simulink model "ElectricalCoupling_testing"  (R2024b)
settings: Solver=FixedStepAuto  StartTime=0.0  StopTime=20  RelTol=1e-3
undefined symbols (not defined in the file): ac4b, c4e6, DiscIntNeverNeededParam
libraries: fl_lib x22, nesl_utility x21, ee_lib x5, simulink x3
(part 1 of 2)
settings Model: Creator=rodri  LastModifiedBy=rodri
settings SolverCC: ConcurrentTasks=on  PositivePriorityOrder=on
settings OptimizationCC: BlockReduction=off  OptimizeBlockIOStorage=off
settings DebuggingCC: TasksWithSamePriorityMsg=none
settings HardwareCC: ProdBitPerLong=64  ProdLongLongMode=on  ProdHWDeviceType=Intel->x86-64 (Linux 64)
settings RTWCC: Description=Simulink Real-Time  SystemTargetFile=slrealtime.tlc  TemplateMakefile=slrealtime_default_tmf  Toolchain=Simulink Real-Time Toolchain  BuildConfiguration=Faster Runs  CodeExecutionProfiling=on  TargetLang=C++  GPUComputeCapability=3.5
settings SimulinkRealTimeTargetCC: InstructionSetFMA=off  LogToMDFFile=off

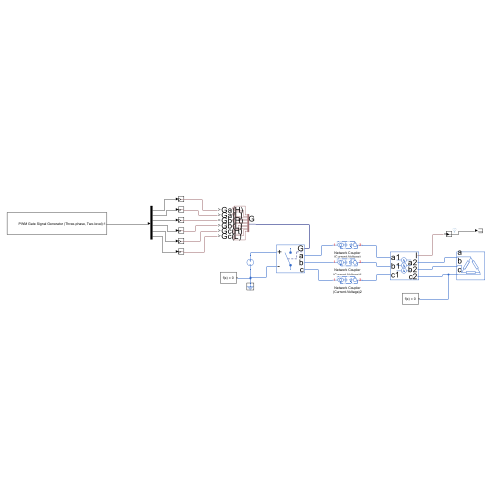
[thumbnail: Simulink's stored preview of the top-level diagram]
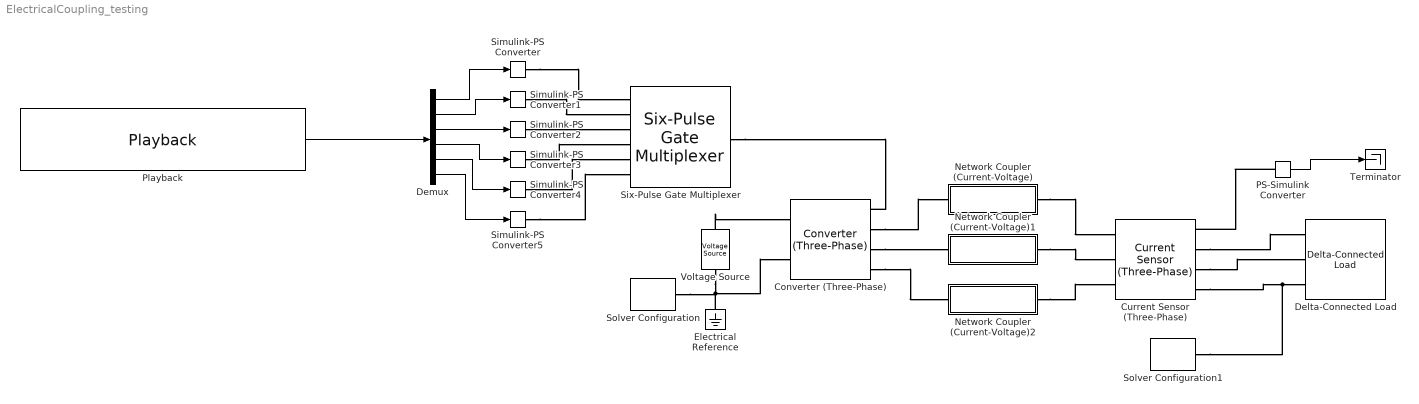
== system ElectricalCoupling_testing ==
  Converter (Three-Phase) : ee_lib/Semiconductors & Converters/Converters/Converter (Three-Phase)  port_option=ee.enum.threePhasePort.expanded  fidelity_option=ee.enum.converters.fidelity.detailed  device_type=ee.enum.converters.switchingdevice.ideal  showThermalPort=false  K=0  Vth=0.5 V  Vgt=1 V  Vgt_off=-1 V  Ih=1 A  Vf=0.8 V  Ron=0.001 Ohm  Rds=0.001 Ohm  Goff=1e-6 1/Ohm  Eon_scalar=22.86e-3 J  Eoff_scalar=17.14e-3 J  Eoff_natural_commutation=10e-3 J  Voff=300 V  Iout_scalar=600 A  onCurrentMeasDelay=0 s  useCurrentFromPreviousCycle=false  useVoltageFromPreviousCycle=false  diode_param=ee.enum.converters.protectiondiode.none  diode_Vf=0.8 V  diode_Ron=0.001 Ohm  diode_Goff=1e-5 1/Ohm  diode_C=50 nF  diode_iRM=-235 A  diode_iF=300 A  diode_idot=-50 A/us  diode_trr_param=ee.enum.converters.diodetrr.trr_factor  diode_trr_factor=3  diode_trr=15 us  diode_Qrr=1500 s*uA  diode_rec_loss_model=ee.enum.diode.reverseRecoveryModel.fixed  diode_ErecVal=0 J  diode_scaleWithIandV=false  diode_ErecMat=zeros(2, 3) J  diode_TjrecVec=[298.15, 398.15] K  diode_IfrecVec=[.1, 1, 10] A  diode_IrecVal=10 A  diode_VrecVal=10 V  diode_tFilter=1 / 1000 / 100 s  thermal_network_parameterization=ee.enum.thermalNetworkTopology.external  Rth=[.08, .5] K/W  Rth_Cauer=[.08, .1, .5] K/W  Rth_Foster=[.08, .14, .22, .16] K/W  thermal_mass_parameterization=ee.enum.thermalNetwork.timeconstant  thermal_mass=[.01, .5] J/K  thermal_mass_Cauer=[.01, .1, .5] J/K  thermal_mass_Foster=[.001, .005, .05, .5] J/K  thermal_time_constant=[.001, .2] s  thermal_time_constant_Cauer=[.001, .1, .2] s  thermal_time_constant_Foster=[7e-05, .0007, .01, .08] s  thermal_mass_initial_temperatures=[25, 25] degC  thermal_mass_initial_temperatures_Cauer=[25, 25, 25] degC  junction_thermal_mass=0.01 J/K  Tvec_initial_Foster=[25, 25, 25, 25] degC  snubber_type=ee.enum.converters.snubber.exclude  Cs=1e-7 F  Rs=0.1 Ohm  Vce_loss=[0, 150, 300] V
      settings: InternalSimscapePortConfiguration="{\"Bottom\":[],\"Left\":[{\"id\":\"G\",\"label\":\"G\",\"type\":\"foundation.electrical.twelve_phase\"},{\"id\":\"a\",\"label\":\"a\",\"type\":\"foundation.electrical.electrical\"},{\"id\":\"b\",\"label\":\"b\",\"type\":\"foundation.electrical.electrical\"},{\"id\":\"c\",\"label\":\"c\",\"type\":\"foundation.electrical.electrical\"}],\"Right\":[{\"id\":\"p\",\"label\":\"+\",\"type\":\"foundation.electrical.electrical\"},{\"id\":\"n\",\"label\":\"-\",\"type\":\"foundation.electrical.electrical\"}],\"Top\":[]}"
  Current Sensor (Three-Phase) : ee_lib/Sensors & Transducers/Current Sensor (Three-Phase)
      settings: InternalSimscapePortConfiguration="{\"Bottom\":[],\"Left\":[{\"id\":\"a1\",\"label\":\"a1\",\"type\":\"foundation.electrical.electrical\"},{\"id\":\"b1\",\"label\":\"b1\",\"type\":\"foundation.electrical.electrical\"},{\"id\":\"c1\",\"label\":\"c1\",\"type\":\"foundation.electrical.electrical\"}],\"Right\":[{\"id\":\"I_output\",\"label\":\"I\",\"type\":\"output\"},{\"id\":\"a2\",\"label\":\"a2\",\"type\":\"foundation.electrical.electrical\"},{\"id\":\"b2\",\"label\":\"b2\",\"type\":\"foundation.electrical.electrical\"},{\"id\":\"c2\",\"label\":\"c2\",\"type\":\"foundation.electrical.electrical\"}],\"Top\":[]}"
  Delta-Connected Load : ee_lib/Passive/RLC Assemblies/Delta-Connected Load  port_option=ee.enum.threePhasePort.expanded  parameterization=ee.enum.rlc.parameterization.ratedpower  component_structure=ee.enum.rlc.structure.R  component_structure_PQ=ee.enum.rlc.structure.SeriesRL  R=1 Ohm  L=1e-3 H  C=1e-6 F  VRated=380 V  FRated=60 Hz  P=10e3 W  Qpos=1e3 A*V  Qneg=-1e2 A*V  R_parasitic=0 Ohm  G_parasitic=0 1/Ohm  R_parasitic_PQ=0 Ohm  G_parasitic_PQ=0 1/Ohm  Vmag0=0 V  Vang0=0 deg  Freq0=60 Hz  IL_specify=off  IL_priority=High  IL=[0, 0, 0] A  IL_nominal_specify=off  IL_nominal_value=1  IL_nominal_unit=A  VC_specify=off  VC_priority=High  VC=[0, 0, 0] V  VC_nominal_specify=off  VC_nominal_value=1  VC_nominal_unit=V
      settings: InternalSimscapePortConfiguration="{\"Bottom\":[],\"Left\":[{\"id\":\"a\",\"label\":\"a\",\"type\":\"foundation.electrical.electrical\"},{\"id\":\"b\",\"label\":\"b\",\"type\":\"foundation.electrical.electrical\"},{\"id\":\"c\",\"label\":\"c\",\"type\":\"foundation.electrical.electrical\"}],\"Right\":[],\"Top\":[]}"
  Demux : Demux  Outputs=6
  Electrical Reference : fl_lib/Electrical/Electrical Elements/Electrical Reference
  Network Coupler (Current-Voltage) : Subsystem  mask(Network Coupler (Current-Voltage)){}
      mask init:
      | % Icon
      | key = 'Simscape.NetworkCouplers.ElectricalCurrentVoltage';
      | foundation.internal.couplers.updateIcon(gcb,'currentVoltageSource.svg',key)
      settings: OpenFcn=open_system(gcbh,'force')
      mask Help: web([docroot '/simscape/ref/networkcouplercurrentvoltage.html'])
      mask Display:
      | color('red');
      | port_label('LConn', 1,'1')
      | port_label('RConn', 1,'2')
  Network Coupler (Current-Voltage)1 : Subsystem  mask(Network Coupler (Current-Voltage)){}
      mask init:
      | % Icon
      | key = 'Simscape.NetworkCouplers.ElectricalCurrentVoltage';
      | foundation.internal.couplers.updateIcon(gcb,'currentVoltageSource.svg',key)
      settings: OpenFcn=open_system(gcbh,'force')
      mask Help: web([docroot '/simscape/ref/networkcouplercurrentvoltage.html'])
      mask Display:
      | color('red');
      | port_label('LConn', 1,'1')
      | port_label('RConn', 1,'2')
  Network Coupler (Current-Voltage)2 : Subsystem  mask(Network Coupler (Current-Voltage)){}
      mask init:
      | % Icon
      | key = 'Simscape.NetworkCouplers.ElectricalCurrentVoltage';
      | foundation.internal.couplers.updateIcon(gcb,'currentVoltageSource.svg',key)
      settings: OpenFcn=open_system(gcbh,'force')
      mask Help: web([docroot '/simscape/ref/networkcouplercurrentvoltage.html'])
      mask Display:
      | color('red');
      | port_label('LConn', 1,'1')
      | port_label('RConn', 1,'2')
  PS-Simulink Converter : nesl_utility/PS-Simulink Converter  PhysicalDomain=network_engine_domain  SubClassName=ps_output  LeftPortType=input  RightPortType=output  PseudoPeriodic=off  Frequencies=[]  VectorFormat=inherit  Unit=inherit  AffineConversion=off
  Playback : Playback  NumPorts=1  PartName=31bf6123-c4e6-46bc-ac4b-6301b38411a2
  Simulink-PS Converter{,1..5} (6 alike) : nesl_utility/Simulink-PS Converter  PhysicalDomain=network_engine_domain  SubClassName=ps_input  LeftPortType=input  RightPortType=output  PseudoPeriodic=off  Frequencies=[]  NoiseDistribution=none  NoiseParameters=[]  Unit=1  AffineConversion=off  FilteringAndDerivatives=provide  SimscapeFilterOrder=1  InputFilterTimeConstant=0.001  UdotUserProvided=0
  Six-Pulse Gate Multiplexer : ee_lib/Semiconductors & Converters/Converters/Six-Pulse Gate Multiplexer  port_option=ee.enum.controlport.ps
  Solver Configuration : nesl_utility/Solver Configuration  PhysicalDomain=network_engine_domain  SubClassName=solver  LeftPortType=input  RightPortType=generic  Tones=[]  Harmonics=[]  SimulateNoise=off  Profile=off  UseLocalSampling=off  EnableSwitchedLinearOptims=on  FrequencyDomain=off  UseCCode=off  RelTol=0.001  AbsTol=0.001  MinStep=1e-09  ToWorkspace=off  RevertToSquareIcSolve=off  NumHomotopyIterations=100  PhasorMode=off  PhasorModeNumHarmonics=1  ConsistencySolver=NEWTON_XTOL_AFTER_FTOL  IndexReductionMethod=DerivativeReplacement  DoDC=off  ResidualTolerance=1e-09  ConsistencyTolSource=GLOBAL  ConsistencyAbsTol=0.001  ConsistencyRelTol=0.001  ConsistencyTolFactor=0.001  UseLocalSolver=off  LocalSolverChoice=NE_BACKWARD_EULER_ADVANCER  ResolveIndetEquations=on  FunctionEvalNumThread=1  LocalSolverSampleTime=0.001  DoFixedCost=off  MaxNonlinIter=3  MaxModeIter=2  ComputeImpulses=off  ImpulseIterations=2  LinearAlgebra=auto  LinearAlgebraNumThread=0  EquationFormulation=NE_TIME_EF  DelaysMemoryBudget=1024  AutomaticFiltering=on  FilteringTimeConstant=0.001  PartitionStorageMethod=AS_NEEDED  PartitionMemoryBudget=1024  PartitionMethod=ROBUST  MultibodyUseLocalSolver=off  MultibodyLocalSolverChoice=ODE1  MultibodyLocalSolverSampleTime=0.001
  Solver Configuration1 : nesl_utility/Solver Configuration  PhysicalDomain=network_engine_domain  SubClassName=solver  LeftPortType=input  RightPortType=generic  Tones=[]  Harmonics=[]  SimulateNoise=off  Profile=off  UseLocalSampling=off  EnableSwitchedLinearOptims=on  FrequencyDomain=off  UseCCode=off  RelTol=0.001  AbsTol=0.001  MinStep=1e-09  ToWorkspace=off  RevertToSquareIcSolve=off  NumHomotopyIterations=100  PhasorMode=off  PhasorModeNumHarmonics=1  ConsistencySolver=NEWTON_XTOL_AFTER_FTOL  IndexReductionMethod=DerivativeReplacement  DoDC=off  ResidualTolerance=1e-09  ConsistencyTolSource=GLOBAL  ConsistencyAbsTol=0.001  ConsistencyRelTol=0.001  ConsistencyTolFactor=0.001  UseLocalSolver=off  LocalSolverChoice=NE_BACKWARD_EULER_ADVANCER  ResolveIndetEquations=on  FunctionEvalNumThread=1  LocalSolverSampleTime=0.001  DoFixedCost=off  MaxNonlinIter=3  MaxModeIter=2  ComputeImpulses=off  ImpulseIterations=2  LinearAlgebra=auto  LinearAlgebraNumThread=0  EquationFormulation=NE_TIME_EF  DelaysMemoryBudget=1024  AutomaticFiltering=on  FilteringTimeConstant=0.001  PartitionStorageMethod=AS_NEEDED  PartitionMemoryBudget=1024  PartitionMethod=ROBUST  MultibodyUseLocalSolver=off  MultibodyLocalSolverChoice=ODE1  MultibodyLocalSolverSampleTime=0.001
  Terminator : Terminator
  Voltage Source : ee_lib/Sources/Voltage Source  dc_voltage=380 V  ac_voltage=0 V  ac_shift=0 rad  ac_frequency=60 Hz  noise_mode=ee.enum.sources.noise.Disabled  PSD=0 V^2/Hz  sample_time=1e-3 s  repeatability=ee.enum.sources.repeatability.NotRepeatable  user_seed=0  auto_seed=3499211588  i_specify=off  i_priority=None  i=0 A  i_nominal_specify=off  i_nominal_value=1  i_nominal_unit=A  v_specify=off  v_priority=None  v=0 V  v_nominal_specify=off  v_nominal_value=1  v_nominal_unit=V
  wires:
  Demux/1 -> Simulink-PS Converter/1
  Demux/2 -> Simulink-PS Converter1/1
  Demux/3 -> Simulink-PS Converter2/1
  Demux/4 -> Simulink-PS Converter3/1
  Demux/5 -> Simulink-PS Converter4/1
  Demux/6 -> Simulink-PS Converter5/1
  Playback/1 -> Demux/1
  PS-Simulink Converter/1 -> Terminator/1
  connections:
  Simulink-PS Converter2/RConn1 -- Six-Pulse Gate Multiplexer/LConn3
  Simulink-PS Converter1/RConn1 -- Six-Pulse Gate Multiplexer/LConn2
  Simulink-PS Converter3/RConn1 -- Six-Pulse Gate Multiplexer/LConn4
  Simulink-PS Converter/RConn1 -- Six-Pulse Gate Multiplexer/LConn1
  Simulink-PS Converter4/RConn1 -- Six-Pulse Gate Multiplexer/LConn5
  Simulink-PS Converter5/RConn1 -- Six-Pulse Gate Multiplexer/LConn6
  Six-Pulse Gate Multiplexer/RConn1 -- Converter (Three-Phase)/LConn1
  Voltage Source/LConn1 -- Converter (Three-Phase)/RConn1
  Voltage Source/RConn1 -- Solver Configuration/RConn1 -- Electrical Reference/LConn1 -- Converter (Three-Phase)/RConn2
  Current Sensor (Three-Phase)/RConn2 -- Delta-Connected Load/LConn1
  PS-Simulink Converter/LConn1 -- Current Sensor (Three-Phase)/RConn1
  Converter (Three-Phase)/LConn2 -- Network Coupler (Current-Voltage)/LConn1
  Network Coupler (Current-Voltage)/RConn1 -- Current Sensor (Three-Phase)/LConn1
  Network Coupler (Current-Voltage)1/RConn1 -- Current Sensor (Three-Phase)/LConn2
  Converter (Three-Phase)/LConn3 -- Network Coupler (Current-Voltage)1/LConn1
  Converter (Three-Phase)/LConn4 -- Network Coupler (Current-Voltage)2/LConn1
  Network Coupler (Current-Voltage)2/RConn1 -- Current Sensor (Three-Phase)/LConn3
  Current Sensor (Three-Phase)/RConn4 -- Solver Configuration1/RConn1 -- Delta-Connected Load/LConn3
  Current Sensor (Three-Phase)/RConn3 -- Delta-Connected Load/LConn2

== system ElectricalCoupling_testing/Network Coupler (Current-Voltage) ==
  note: Connect Port 1 to the network
      | with the smaller sample time, or
      | the network running variable step.
  note: Uncomment rate transition
      | blocks if one or both networks
      | are running fixed step.
  Port 1 Interface : Subsystem  mask(Network Coupler (Current-Voltage) Port 1 Interface){samplingType=Variable step at ports 1 and 2, ts=1e-3, h1=0.0002, h2=0.001, predictionDiscreteToContinuous=off, smoothingContinuousToDiscrete=off, predictionSlowToFast=off, smoothingFastToSlow=off, nSmooth=1, tsSmoothing=0.01, tsMax=0.005, tau=0.001, i0=0, v0=0}
      mask prompts: samplingType "physmod:simscape:couplers:SimscapeNetworkCouplersLib:SamplingType_MP"; ts "physmod:simscape:couplers:SimscapeNetworkCouplersLib:SeparatorTimeConstants_MP"; h1 "physmod:simscape:couplers:SimscapeNetworkCouplersLib:Port1NetworkDiscreteSampleTimes_MP"; h2 "physmod:simscape:couplers:SimscapeNetworkCouplersLib:Port2NetworkDiscreteSampleTimes_MP"; predictionDiscreteToContinuous "physmod:simscape:couplers:SimscapeNetworkCouplersLib:UsePredictionWhenConnectingFixedStepToVariableStep_MP"; smoothingContinuousToDiscrete "physmod:simscape:couplers:SimscapeNetworkCouplersLib:UseSmoothingWhenConnectingVariableStepToFixedStep_MP"; predictionSlowToFast "physmod:simscape:couplers:SimscapeNetworkCouplersLib:UsePredictionWhenConnectingSlowToFastSampleTimes_MP"; smoothingFastToSlow "physmod:simscape:couplers:SimscapeNetworkCouplersLib:UseSmoothingWhenConnectingFastToSlowSampleTimes_MP"; nSmooth "physmod:simscape:couplers:SimscapeNetworkCouplersLib:NumberOfSamplesOverWhichToSmooth_MP"; tsSmoothing "physmod:simscape:couplers:SimscapeNetworkCouplersLib:SmoothingTimeConstants_MP"; tsMax "physmod:simscape:couplers:SimscapeNetworkCouplersLib:CalculatedFastestTrackableTimeConstants_MP"; tau "physmod:simscape:couplers:SimscapeNetworkCouplersLib:CalculatedFilterTimeConstants_MP"; i0 "physmod:simscape:couplers:SimscapeNetworkCouplersLib:InitialCurrentA_MP"; v0 "physmod:simscape:couplers:SimscapeNetworkCouplersLib:InitialVoltageV_MP"
      mask help: physmod:simscape:couplers:SimscapeNetworkCouplersLib:NetworkCouplerCurrentVoltagePort1Interface_MD
      mask init:
      | % Fixed step sample time value check
      | foundation.internal.couplers.checkSampleTimes(gcb,h1,h2);
      | 
      | % Derived parameters
      | [tau,tsMax] = foundation.internal.couplers.electrical.derivedParamsSources(gcb,ts,h1,h2);
      settings: PortSchema="{\"entries\":[{\"content\":{\"sides\":[{\"content\":{\"connectorIds\":[\"LConn1\"]},\"type\":\"ConnectorPlacement.EquallySpacedRectSide\",\"uuid\":\"a6d4a9fd-b5aa-40dc-ab7e-2b646b9b57bc\"},{\"content\":{\"connectorIds\":[\"Out1\",\"In1\"],\"side\":\"RIGHT\"},\"type\":\"ConnectorPlacement.EquallySpacedRectSide\",\"uuid\":\"31bb6273-5b9b-48d0-a1a2-6fbacb979b97\"},{\"content\":{\"connectorIds\":[],\"side\":\"TOP\"},\"type\":\"ConnectorPlacement.EquallySpacedRectSide\",\"uuid\":\"0f7afab2-4481-486c-9ad0-2b42c5b091a4\"}]},\"type\":\"ConnectorPlacement.EquallySpacedConnector\",\"uuid\":\"a98e47aa-cbfd-441a-b14c-c9ea515c056e\"}],\"packageUris\":[\"http://schema.mathworks.com/mf0/Connector/R2020b\"],\"version\":\"1.0\"}"
      mask Help: web([docroot '/simscape/ref/networkcouplercurrentvoltage.html'])
      mask TypeOptions samplingType: physmod:simscape:couplers:SimscapeNetworkCouplersLib:VariableStepAtPorts1And2_PV | physmod:simscape:couplers:SimscapeNetworkCouplersLib:VariableStepAtPort1AndFixedStepAtPort2_PV | physmod:simscape:couplers:SimscapeNetworkCouplersLib:FixedStepBothPortsWithCommonSampleTime_PV | physmod:simscape:couplers:SimscapeNetworkCouplersLib:FixedStepBothPortsWithFasterSamplingAtPort1_PV
      mask Callback samplingType: foundation.internal.couplers.electrical.parameterVisibilitiesSources(gcb)
      mask Callback predictionDiscreteToContinuous: foundation.internal.couplers.electrical.parameterVisibilitiesSources(gcb)
      mask Callback smoothingContinuousToDiscrete: foundation.internal.couplers.electrical.parameterVisibilitiesSources(gcb)
      mask Callback predictionSlowToFast: foundation.internal.couplers.electrical.parameterVisibilitiesSources(gcb)
      mask Callback smoothingFastToSlow: foundation.internal.couplers.electrical.parameterVisibilitiesSources(gcb)
      mask DialogControl Main Prompt: physmod:simscape:couplers:SimscapeNetworkCouplersLib:tab_Main
      mask DialogControl samplingType Prompt: Sampling type
      mask DialogControl ts Prompt: Separator time constant (s)
      mask DialogControl h1 Prompt: Port 1 network discrete sample time (s)
      mask DialogControl h2 Prompt: Port 2 network discrete sample time (s)
      mask DialogControl predictionDiscreteToContinuous Prompt: Use prediction when connecting fixed step to variable step
      mask DialogControl smoothingContinuousToDiscrete Prompt: Use smoothing when connecting variable step to fixed step
      mask DialogControl predictionSlowToFast Prompt: Use prediction when connecting slow to fast sample times
      mask DialogControl smoothingFastToSlow Prompt: Use smoothing when connecting fast to slow sample times
      mask DialogControl nSmooth Prompt: Number of samples over which to smooth
      mask DialogControl tsSmoothing Prompt: Smoothing time constant (s)
      mask DialogControl Analysis Prompt: physmod:simscape:couplers:SimscapeNetworkCouplersLib:tab_Analysis
      mask DialogControl tsMax Prompt: Calculated fastest trackable time constant (s)
      mask DialogControl tau Prompt: Calculated filter time constant (s)
      mask DialogControl updateRecommendations Prompt: physmod:simscape:couplers:SimscapeNetworkCouplersLib:button_Update
      mask DialogControl updateRecommendations Callback: foundation.internal.couplers.electrical.analysisSources(gcb);
      mask DialogControl InitialConditions Prompt: physmod:simscape:couplers:SimscapeNetworkCouplersLib:tab_InitialConditions
      mask DialogControl i0 Prompt: Initial current (A)
      mask DialogControl v0 Prompt: Initial voltage (V)
  Port 2 Interface : Subsystem  mask(Network Coupler (Current-Voltage) Port 2 Interface){}
      mask help: physmod:simscape:couplers:SimscapeNetworkCouplersLib:NetworkCouplerCurrentVoltagePort2Interface_MD
      settings: PortSchema="{\"entries\":[{\"content\":{\"sides\":[{\"content\":{\"connectorIds\":[\"In1\",\"Out1\"]},\"type\":\"ConnectorPlacement.EquallySpacedRectSide\",\"uuid\":\"5a4c1550-e77d-42df-bf3e-b81963920de7\"},{\"content\":{\"connectorIds\":[\"RConn1\"],\"side\":\"RIGHT\"},\"type\":\"ConnectorPlacement.EquallySpacedRectSide\",\"uuid\":\"3fd730f7-5937-4563-a365-595aaae9027b\"},{\"content\":{\"connectorIds\":[],\"side\":\"TOP\"},\"type\":\"ConnectorPlacement.EquallySpacedRectSide\",\"uuid\":\"c16e04e4-26e8-4fd6-98d3-59adbef44c0d\"}]},\"type\":\"ConnectorPlacement.EquallySpacedConnector\",\"uuid\":\"5588d8d0-d459-45fe-a303-1ca6654e99d0\"}],\"packageUris\":[\"http://schema.mathworks.com/mf0/Connector/R2020b\"],\"version\":\"1.0\"}"
      mask Help: web([docroot '/simscape/ref/networkcouplercurrentvoltage.html'])
  Rate transition (fast-to-slow) : RateTransition  Commented=through  Integrity=off
  Rate transition (slow-to-fast) : RateTransition  Commented=through  Integrity=off
  1 : PMIOPort  Side=Left
  2 : PMIOPort  Port=2  Side=Right
  wires:
  Rate transition (slow-to-fast)/1 -> Port 1 Interface/1(current)
  Port 2 Interface/1(current) -> Rate transition (slow-to-fast)/1
  Rate transition (fast-to-slow)/1 -> Port 2 Interface/1(voltage)
  Port 1 Interface/1(voltage) -> Rate transition (fast-to-slow)/1
  connections:
  1/RConn1 -- Port 1 Interface/LConn1
  2/RConn1 -- Port 2 Interface/RConn1

== system ElectricalCoupling_testing/Network Coupler (Current-Voltage)1 ==
  note: Uncomment rate transition
      | blocks if one or both networks
      | are running fixed step.
  note: Connect Port 1 to the network
      | with the smaller sample time, or
      | the network running variable step.
  Port 1 Interface : Subsystem  mask(Network Coupler (Current-Voltage) Port 1 Interface){samplingType=Variable step at ports 1 and 2, ts=1e-3, h1=0.0002, h2=0.001, predictionDiscreteToContinuous=off, smoothingContinuousToDiscrete=off, predictionSlowToFast=off, smoothingFastToSlow=off, nSmooth=1, tsSmoothing=0.01, tsMax=0.005, tau=0.001, i0=0, v0=0}
      mask prompts: samplingType "physmod:simscape:couplers:SimscapeNetworkCouplersLib:SamplingType_MP"; ts "physmod:simscape:couplers:SimscapeNetworkCouplersLib:SeparatorTimeConstants_MP"; h1 "physmod:simscape:couplers:SimscapeNetworkCouplersLib:Port1NetworkDiscreteSampleTimes_MP"; h2 "physmod:simscape:couplers:SimscapeNetworkCouplersLib:Port2NetworkDiscreteSampleTimes_MP"; predictionDiscreteToContinuous "physmod:simscape:couplers:SimscapeNetworkCouplersLib:UsePredictionWhenConnectingFixedStepToVariableStep_MP"; smoothingContinuousToDiscrete "physmod:simscape:couplers:SimscapeNetworkCouplersLib:UseSmoothingWhenConnectingVariableStepToFixedStep_MP"; predictionSlowToFast "physmod:simscape:couplers:SimscapeNetworkCouplersLib:UsePredictionWhenConnectingSlowToFastSampleTimes_MP"; smoothingFastToSlow "physmod:simscape:couplers:SimscapeNetworkCouplersLib:UseSmoothingWhenConnectingFastToSlowSampleTimes_MP"; nSmooth "physmod:simscape:couplers:SimscapeNetworkCouplersLib:NumberOfSamplesOverWhichToSmooth_MP"; tsSmoothing "physmod:simscape:couplers:SimscapeNetworkCouplersLib:SmoothingTimeConstants_MP"; tsMax "physmod:simscape:couplers:SimscapeNetworkCouplersLib:CalculatedFastestTrackableTimeConstants_MP"; tau "physmod:simscape:couplers:SimscapeNetworkCouplersLib:CalculatedFilterTimeConstants_MP"; i0 "physmod:simscape:couplers:SimscapeNetworkCouplersLib:InitialCurrentA_MP"; v0 "physmod:simscape:couplers:SimscapeNetworkCouplersLib:InitialVoltageV_MP"
      mask help: physmod:simscape:couplers:SimscapeNetworkCouplersLib:NetworkCouplerCurrentVoltagePort1Interface_MD
      mask init: same as ElectricalCoupling_testing/Network Coupler (Current-Voltage)/Port 1 Interface
      settings: PortSchema="{\"entries\":[{\"content\":{\"sides\":[{\"content\":{\"connectorIds\":[\"LConn1\"]},\"type\":\"ConnectorPlacement.EquallySpacedRectSide\",\"uuid\":\"a6d4a9fd-b5aa-40dc-ab7e-2b646b9b57bc\"},{\"content\":{\"connectorIds\":[\"Out1\",\"In1\"],\"side\":\"RIGHT\"},\"type\":\"ConnectorPlacement.EquallySpacedRectSide\",\"uuid\":\"31bb6273-5b9b-48d0-a1a2-6fbacb979b97\"},{\"content\":{\"connectorIds\":[],\"side\":\"TOP\"},\"type\":\"ConnectorPlacement.EquallySpacedRectSide\",\"uuid\":\"0f7afab2-4481-486c-9ad0-2b42c5b091a4\"}]},\"type\":\"ConnectorPlacement.EquallySpacedConnector\",\"uuid\":\"a98e47aa-cbfd-441a-b14c-c9ea515c056e\"}],\"packageUris\":[\"http://schema.mathworks.com/mf0/Connector/R2020b\"],\"version\":\"1.0\"}"
      mask Help: web([docroot '/simscape/ref/networkcouplercurrentvoltage.html'])
      mask TypeOptions samplingType: physmod:simscape:couplers:SimscapeNetworkCouplersLib:VariableStepAtPorts1And2_PV | physmod:simscape:couplers:SimscapeNetworkCouplersLib:VariableStepAtPort1AndFixedStepAtPort2_PV | physmod:simscape:couplers:SimscapeNetworkCouplersLib:FixedStepBothPortsWithCommonSampleTime_PV | physmod:simscape:couplers:SimscapeNetworkCouplersLib:FixedStepBothPortsWithFasterSamplingAtPort1_PV
      mask Callback samplingType: foundation.internal.couplers.electrical.parameterVisibilitiesSources(gcb)
      mask Callback predictionDiscreteToContinuous: foundation.internal.couplers.electrical.parameterVisibilitiesSources(gcb)
      mask Callback smoothingContinuousToDiscrete: foundation.internal.couplers.electrical.parameterVisibilitiesSources(gcb)
      mask Callback predictionSlowToFast: foundation.internal.couplers.electrical.parameterVisibilitiesSources(gcb)
      mask Callback smoothingFastToSlow: foundation.internal.couplers.electrical.parameterVisibilitiesSources(gcb)
      mask DialogControl Main Prompt: physmod:simscape:couplers:SimscapeNetworkCouplersLib:tab_Main
      mask DialogControl samplingType Prompt: Sampling type
      mask DialogControl ts Prompt: Separator time constant (s)
      mask DialogControl h1 Prompt: Port 1 network discrete sample time (s)
      mask DialogControl h2 Prompt: Port 2 network discrete sample time (s)
      mask DialogControl predictionDiscreteToContinuous Prompt: Use prediction when connecting fixed step to variable step
      mask DialogControl smoothingContinuousToDiscrete Prompt: Use smoothing when connecting variable step to fixed step
      mask DialogControl predictionSlowToFast Prompt: Use prediction when connecting slow to fast sample times
      mask DialogControl smoothingFastToSlow Prompt: Use smoothing when connecting fast to slow sample times
      mask DialogControl nSmooth Prompt: Number of samples over which to smooth
      mask DialogControl tsSmoothing Prompt: Smoothing time constant (s)
      mask DialogControl Analysis Prompt: physmod:simscape:couplers:SimscapeNetworkCouplersLib:tab_Analysis
      mask DialogControl tsMax Prompt: Calculated fastest trackable time constant (s)
      mask DialogControl tau Prompt: Calculated filter time constant (s)
      mask DialogControl updateRecommendations Prompt: physmod:simscape:couplers:SimscapeNetworkCouplersLib:button_Update
      mask DialogControl updateRecommendations Callback: foundation.internal.couplers.electrical.analysisSources(gcb);
      mask DialogControl InitialConditions Prompt: physmod:simscape:couplers:SimscapeNetworkCouplersLib:tab_InitialConditions
      mask DialogControl i0 Prompt: Initial current (A)
      mask DialogControl v0 Prompt: Initial voltage (V)
  Port 2 Interface : Subsystem  mask(Network Coupler (Current-Voltage) Port 2 Interface){}
      mask help: physmod:simscape:couplers:SimscapeNetworkCouplersLib:NetworkCouplerCurrentVoltagePort2Interface_MD
      settings: PortSchema="{\"entries\":[{\"content\":{\"sides\":[{\"content\":{\"connectorIds\":[\"In1\",\"Out1\"]},\"type\":\"ConnectorPlacement.EquallySpacedRectSide\",\"uuid\":\"5a4c1550-e77d-42df-bf3e-b81963920de7\"},{\"content\":{\"connectorIds\":[\"RConn1\"],\"side\":\"RIGHT\"},\"type\":\"ConnectorPlacement.EquallySpacedRectSide\",\"uuid\":\"3fd730f7-5937-4563-a365-595aaae9027b\"},{\"content\":{\"connectorIds\":[],\"side\":\"TOP\"},\"type\":\"ConnectorPlacement.EquallySpacedRectSide\",\"uuid\":\"c16e04e4-26e8-4fd6-98d3-59adbef44c0d\"}]},\"type\":\"ConnectorPlacement.EquallySpacedConnector\",\"uuid\":\"5588d8d0-d459-45fe-a303-1ca6654e99d0\"}],\"packageUris\":[\"http://schema.mathworks.com/mf0/Connector/R2020b\"],\"version\":\"1.0\"}"
      mask Help: web([docroot '/simscape/ref/networkcouplercurrentvoltage.html'])
  Rate transition (fast-to-slow) : RateTransition  Commented=through  Integrity=off
  Rate transition (slow-to-fast) : RateTransition  Commented=through  Integrity=off
  1 : PMIOPort  Side=Left
  2 : PMIOPort  Port=2  Side=Right
  wires:
  Port 1 Interface/1(voltage) -> Rate transition (fast-to-slow)/1
  Rate transition (fast-to-slow)/1 -> Port 2 Interface/1(voltage)
  Port 2 Interface/1(current) -> Rate transition (slow-to-fast)/1
  Rate transition (slow-to-fast)/1 -> Port 1 Interface/1(current)
  connections:
  2/RConn1 -- Port 2 Interface/RConn1
  1/RConn1 -- Port 1 Interface/LConn1

== system ElectricalCoupling_testing/Network Coupler (Current-Voltage)2 ==
  note: Connect Port 1 to the network
      | with the smaller sample time, or
      | the network running variable step.
  note: Uncomment rate transition
      | blocks if one or both networks
      | are running fixed step.
  Port 1 Interface : Subsystem  mask(Network Coupler (Current-Voltage) Port 1 Interface){samplingType=Variable step at ports 1 and 2, ts=1e-3, h1=0.0002, h2=0.001, predictionDiscreteToContinuous=off, smoothingContinuousToDiscrete=off, predictionSlowToFast=off, smoothingFastToSlow=off, nSmooth=1, tsSmoothing=0.01, tsMax=0.005, tau=0.001, i0=0, v0=0}
      mask prompts: samplingType "physmod:simscape:couplers:SimscapeNetworkCouplersLib:SamplingType_MP"; ts "physmod:simscape:couplers:SimscapeNetworkCouplersLib:SeparatorTimeConstants_MP"; h1 "physmod:simscape:couplers:SimscapeNetworkCouplersLib:Port1NetworkDiscreteSampleTimes_MP"; h2 "physmod:simscape:couplers:SimscapeNetworkCouplersLib:Port2NetworkDiscreteSampleTimes_MP"; predictionDiscreteToContinuous "physmod:simscape:couplers:SimscapeNetworkCouplersLib:UsePredictionWhenConnectingFixedStepToVariableStep_MP"; smoothingContinuousToDiscrete "physmod:simscape:couplers:SimscapeNetworkCouplersLib:UseSmoothingWhenConnectingVariableStepToFixedStep_MP"; predictionSlowToFast "physmod:simscape:couplers:SimscapeNetworkCouplersLib:UsePredictionWhenConnectingSlowToFastSampleTimes_MP"; smoothingFastToSlow "physmod:simscape:couplers:SimscapeNetworkCouplersLib:UseSmoothingWhenConnectingFastToSlowSampleTimes_MP"; nSmooth "physmod:simscape:couplers:SimscapeNetworkCouplersLib:NumberOfSamplesOverWhichToSmooth_MP"; tsSmoothing "physmod:simscape:couplers:SimscapeNetworkCouplersLib:SmoothingTimeConstants_MP"; tsMax "physmod:simscape:couplers:SimscapeNetworkCouplersLib:CalculatedFastestTrackableTimeConstants_MP"; tau "physmod:simscape:couplers:SimscapeNetworkCouplersLib:CalculatedFilterTimeConstants_MP"; i0 "physmod:simscape:couplers:SimscapeNetworkCouplersLib:InitialCurrentA_MP"; v0 "physmod:simscape:couplers:SimscapeNetworkCouplersLib:InitialVoltageV_MP"
      mask help: physmod:simscape:couplers:SimscapeNetworkCouplersLib:NetworkCouplerCurrentVoltagePort1Interface_MD
      mask init: same as ElectricalCoupling_testing/Network Coupler (Current-Voltage)/Port 1 Interface
      settings: PortSchema="{\"entries\":[{\"content\":{\"sides\":[{\"content\":{\"connectorIds\":[\"LConn1\"]},\"type\":\"ConnectorPlacement.EquallySpacedRectSide\",\"uuid\":\"a6d4a9fd-b5aa-40dc-ab7e-2b646b9b57bc\"},{\"content\":{\"connectorIds\":[\"Out1\",\"In1\"],\"side\":\"RIGHT\"},\"type\":\"ConnectorPlacement.EquallySpacedRectSide\",\"uuid\":\"31bb6273-5b9b-48d0-a1a2-6fbacb979b97\"},{\"content\":{\"connectorIds\":[],\"side\":\"TOP\"},\"type\":\"ConnectorPlacement.EquallySpacedRectSide\",\"uuid\":\"0f7afab2-4481-486c-9ad0-2b42c5b091a4\"}]},\"type\":\"ConnectorPlacement.EquallySpacedConnector\",\"uuid\":\"a98e47aa-cbfd-441a-b14c-c9ea515c056e\"}],\"packageUris\":[\"http://schema.mathworks.com/mf0/Connector/R2020b\"],\"version\":\"1.0\"}"
      mask Help: web([docroot '/simscape/ref/networkcouplercurrentvoltage.html'])
      mask TypeOptions samplingType: physmod:simscape:couplers:SimscapeNetworkCouplersLib:VariableStepAtPorts1And2_PV | physmod:simscape:couplers:SimscapeNetworkCouplersLib:VariableStepAtPort1AndFixedStepAtPort2_PV | physmod:simscape:couplers:SimscapeNetworkCouplersLib:FixedStepBothPortsWithCommonSampleTime_PV | physmod:simscape:couplers:SimscapeNetworkCouplersLib:FixedStepBothPortsWithFasterSamplingAtPort1_PV
      mask Callback samplingType: foundation.internal.couplers.electrical.parameterVisibilitiesSources(gcb)
      mask Callback predictionDiscreteToContinuous: foundation.internal.couplers.electrical.parameterVisibilitiesSources(gcb)
      mask Callback smoothingContinuousToDiscrete: foundation.internal.couplers.electrical.parameterVisibilitiesSources(gcb)
      mask Callback predictionSlowToFast: foundation.internal.couplers.electrical.parameterVisibilitiesSources(gcb)
      mask Callback smoothingFastToSlow: foundation.internal.couplers.electrical.parameterVisibilitiesSources(gcb)
      mask DialogControl Main Prompt: physmod:simscape:couplers:SimscapeNetworkCouplersLib:tab_Main
      mask DialogControl samplingType Prompt: Sampling type
      mask DialogControl ts Prompt: Separator time constant (s)
      mask DialogControl h1 Prompt: Port 1 network discrete sample time (s)
      mask DialogControl h2 Prompt: Port 2 network discrete sample time (s)
      mask DialogControl predictionDiscreteToContinuous Prompt: Use prediction when connecting fixed step to variable step
      mask DialogControl smoothingContinuousToDiscrete Prompt: Use smoothing when connecting variable step to fixed step
      mask DialogControl predictionSlowToFast Prompt: Use prediction when connecting slow to fast sample times
      mask DialogControl smoothingFastToSlow Prompt: Use smoothing when connecting fast to slow sample times
      mask DialogControl nSmooth Prompt: Number of samples over which to smooth
      mask DialogControl tsSmoothing Prompt: Smoothing time constant (s)
      mask DialogControl Analysis Prompt: physmod:simscape:couplers:SimscapeNetworkCouplersLib:tab_Analysis
      mask DialogControl tsMax Prompt: Calculated fastest trackable time constant (s)
      mask DialogControl tau Prompt: Calculated filter time constant (s)
      mask DialogControl updateRecommendations Prompt: physmod:simscape:couplers:SimscapeNetworkCouplersLib:button_Update
      mask DialogControl updateRecommendations Callback: foundation.internal.couplers.electrical.analysisSources(gcb);
      mask DialogControl InitialConditions Prompt: physmod:simscape:couplers:SimscapeNetworkCouplersLib:tab_InitialConditions
      mask DialogControl i0 Prompt: Initial current (A)
      mask DialogControl v0 Prompt: Initial voltage (V)
  Port 2 Interface : Subsystem  mask(Network Coupler (Current-Voltage) Port 2 Interface){}
      mask help: physmod:simscape:couplers:SimscapeNetworkCouplersLib:NetworkCouplerCurrentVoltagePort2Interface_MD
      settings: PortSchema="{\"entries\":[{\"content\":{\"sides\":[{\"content\":{\"connectorIds\":[\"In1\",\"Out1\"]},\"type\":\"ConnectorPlacement.EquallySpacedRectSide\",\"uuid\":\"5a4c1550-e77d-42df-bf3e-b81963920de7\"},{\"content\":{\"connectorIds\":[\"RConn1\"],\"side\":\"RIGHT\"},\"type\":\"ConnectorPlacement.EquallySpacedRectSide\",\"uuid\":\"3fd730f7-5937-4563-a365-595aaae9027b\"},{\"content\":{\"connectorIds\":[],\"side\":\"TOP\"},\"type\":\"ConnectorPlacement.EquallySpacedRectSide\",\"uuid\":\"c16e04e4-26e8-4fd6-98d3-59adbef44c0d\"}]},\"type\":\"ConnectorPlacement.EquallySpacedConnector\",\"uuid\":\"5588d8d0-d459-45fe-a303-1ca6654e99d0\"}],\"packageUris\":[\"http://schema.mathworks.com/mf0/Connector/R2020b\"],\"version\":\"1.0\"}"
      mask Help: web([docroot '/simscape/ref/networkcouplercurrentvoltage.html'])
  Rate transition (fast-to-slow) : RateTransition  Commented=through  Integrity=off
  Rate transition (slow-to-fast) : RateTransition  Commented=through  Integrity=off
  1 : PMIOPort  Side=Left
  2 : PMIOPort  Port=2  Side=Right
  wires:
  Rate transition (slow-to-fast)/1 -> Port 1 Interface/1(current)
  Port 2 Interface/1(current) -> Rate transition (slow-to-fast)/1
  Rate transition (fast-to-slow)/1 -> Port 2 Interface/1(voltage)
  Port 1 Interface/1(voltage) -> Rate transition (fast-to-slow)/1
  connections:
  1/RConn1 -- Port 1 Interface/LConn1
  2/RConn1 -- Port 2 Interface/RConn1

== system ElectricalCoupling_testing/Network Coupler (Current-Voltage)/Port 1 Interface ==
  current : Inport
  Controlled Current Source : fl_lib/Electrical/Electrical Sources/Controlled Current Source
  Electrical Reference : fl_lib/Electrical/Electrical Elements/Electrical Reference
  Electrical Reference1 : fl_lib/Electrical/Electrical Elements/Electrical Reference
  Interface : Subsystem  Variant=on  VariantControlMode=label  VariantControl=Variant1  LabelModeActiveChoice=Continuous
      settings: PortSchema="{\"entries\":[{\"content\":{\"sides\":[{\"content\":{\"connectorIds\":[\"In1\",\"Out2\"]},\"type\":\"ConnectorPlacement.EquallySpacedRectSide\",\"uuid\":\"aa56821c-7799-44e3-b228-553c5b43a68d\"},{\"content\":{\"connectorIds\":[\"In2\",\"Out1\"],\"side\":\"RIGHT\"},\"type\":\"ConnectorPlacement.EquallySpacedRectSide\",\"uuid\":\"8658dee5-55e2-4f33-bdec-e6600ce27fc1\"},{\"content\":{\"connectorIds\":[],\"side\":\"TOP\"},\"type\":\"ConnectorPlacement.EquallySpacedRectSide\",\"uuid\":\"2effe9c6-8e61-4f0c-a39b-329d9ffc707d\"}]},\"type\":\"ConnectorPlacement.EquallySpacedConnector\",\"uuid\":\"c8fc8444-dfc7-49a5-9550-b957635f7d8f\"}],\"packageUris\":[\"http://schema.mathworks.com/mf0/Connector/R2020b\"],\"version\":\"1.0\"}"
  Ip : nesl_utility/Simulink-PS Converter  PhysicalDomain=network_engine_domain  SubClassName=ps_input  LeftPortType=input  RightPortType=output  PseudoPeriodic=off  Frequencies=[]  NoiseDistribution=none  NoiseParameters=[]  Unit=A  AffineConversion=off  FilteringAndDerivatives=zero  SimscapeFilterOrder=1  InputFilterTimeConstant=0.001  UdotUserProvided=1
  Voltage Sensor : fl_lib/Electrical/Electrical Sensors/Voltage Sensor
  Vp : nesl_utility/PS-Simulink Converter  PhysicalDomain=network_engine_domain  SubClassName=ps_output  LeftPortType=input  RightPortType=output  PseudoPeriodic=off  Frequencies=[]  VectorFormat=1-D array  Unit=V  AffineConversion=off
  1 : PMIOPort  Side=Left
  voltage : Outport
  wires:
  Interface/2(through1) -> Ip/1
  Vp/1 -> Interface/1(across1)
  current/1 -> Interface/2(through2)
  Interface/1(across2) -> voltage/1
  connections:
  Electrical Reference1/LConn1 -- Voltage Sensor/RConn2
  Ip/RConn1 -- Controlled Current Source/RConn1
  Voltage Sensor/RConn1 -- Vp/LConn1
  Controlled Current Source/LConn1 -- Electrical Reference/LConn1
  Voltage Sensor/LConn1 -- 1/RConn1 -- Controlled Current Source/RConn2

== system ElectricalCoupling_testing/Network Coupler (Current-Voltage)/Port 2 Interface ==
  voltage : Inport
  Controlled Voltage Source : fl_lib/Electrical/Electrical Sources/Controlled Voltage Source
  Current Sensor : fl_lib/Electrical/Electrical Sensors/Current Sensor
  Electrical Reference : fl_lib/Electrical/Electrical Elements/Electrical Reference
  In : nesl_utility/PS-Simulink Converter  PhysicalDomain=network_engine_domain  SubClassName=ps_output  LeftPortType=input  RightPortType=output  PseudoPeriodic=off  Frequencies=[]  VectorFormat=1-D array  Unit=A  AffineConversion=off
  Vn : nesl_utility/Simulink-PS Converter  PhysicalDomain=network_engine_domain  SubClassName=ps_input  LeftPortType=input  RightPortType=output  PseudoPeriodic=off  Frequencies=[]  NoiseDistribution=none  NoiseParameters=[]  Unit=V  AffineConversion=off  FilteringAndDerivatives=zero  SimscapeFilterOrder=1  InputFilterTimeConstant=0.001  UdotUserProvided=1
  2 : PMIOPort  Side=Right
  current : Outport
  wires:
  voltage/1 -> Vn/1
  In/1 -> current/1
  connections:
  2/RConn1 -- Current Sensor/LConn1
  Vn/RConn1 -- Controlled Voltage Source/RConn1
  Current Sensor/RConn2 -- Controlled Voltage Source/LConn1
  Electrical Reference/LConn1 -- Controlled Voltage Source/RConn2
  Current Sensor/RConn1 -- In/LConn1

== system ElectricalCoupling_testing/Network Coupler (Current-Voltage)1/Port 1 Interface ==
  current : Inport
  Controlled Current Source : fl_lib/Electrical/Electrical Sources/Controlled Current Source
  Electrical Reference : fl_lib/Electrical/Electrical Elements/Electrical Reference
  Electrical Reference1 : fl_lib/Electrical/Electrical Elements/Electrical Reference
  Interface : Subsystem  Variant=on  VariantControlMode=label  VariantControl=Variant1  LabelModeActiveChoice=Continuous
      settings: PortSchema="{\"entries\":[{\"content\":{\"sides\":[{\"content\":{\"connectorIds\":[\"In1\",\"Out2\"]},\"type\":\"ConnectorPlacement.EquallySpacedRectSide\",\"uuid\":\"aa56821c-7799-44e3-b228-553c5b43a68d\"},{\"content\":{\"connectorIds\":[\"In2\",\"Out1\"],\"side\":\"RIGHT\"},\"type\":\"ConnectorPlacement.EquallySpacedRectSide\",\"uuid\":\"8658dee5-55e2-4f33-bdec-e6600ce27fc1\"},{\"content\":{\"connectorIds\":[],\"side\":\"TOP\"},\"type\":\"ConnectorPlacement.EquallySpacedRectSide\",\"uuid\":\"2effe9c6-8e61-4f0c-a39b-329d9ffc707d\"}]},\"type\":\"ConnectorPlacement.EquallySpacedConnector\",\"uuid\":\"c8fc8444-dfc7-49a5-9550-b957635f7d8f\"}],\"packageUris\":[\"http://schema.mathworks.com/mf0/Connector/R2020b\"],\"version\":\"1.0\"}"
  Ip : nesl_utility/Simulink-PS Converter  PhysicalDomain=network_engine_domain  SubClassName=ps_input  LeftPortType=input  RightPortType=output  PseudoPeriodic=off  Frequencies=[]  NoiseDistribution=none  NoiseParameters=[]  Unit=A  AffineConversion=off  FilteringAndDerivatives=zero  SimscapeFilterOrder=1  InputFilterTimeConstant=0.001  UdotUserProvided=1
  Voltage Sensor : fl_lib/Electrical/Electrical Sensors/Voltage Sensor
  Vp : nesl_utility/PS-Simulink Converter  PhysicalDomain=network_engine_domain  SubClassName=ps_output  LeftPortType=input  RightPortType=output  PseudoPeriodic=off  Frequencies=[]  VectorFormat=1-D array  Unit=V  AffineConversion=off
  1 : PMIOPort  Side=Left
  voltage : Outport
  wires:
  Interface/1(across2) -> voltage/1
  current/1 -> Interface/2(through2)
  Vp/1 -> Interface/1(across1)
  Interface/2(through1) -> Ip/1
  connections:
  Controlled Current Source/RConn2 -- 1/RConn1 -- Voltage Sensor/LConn1
  Controlled Current Source/LConn1 -- Electrical Reference/LConn1
  Voltage Sensor/RConn1 -- Vp/LConn1
  Ip/RConn1 -- Controlled Current Source/RConn1
  Electrical Reference1/LConn1 -- Voltage Sensor/RConn2

== system ElectricalCoupling_testing/Network Coupler (Current-Voltage)1/Port 2 Interface ==
  voltage : Inport
  Controlled Voltage Source : fl_lib/Electrical/Electrical Sources/Controlled Voltage Source
  Current Sensor : fl_lib/Electrical/Electrical Sensors/Current Sensor
  Electrical Reference : fl_lib/Electrical/Electrical Elements/Electrical Reference
  In : nesl_utility/PS-Simulink Converter  PhysicalDomain=network_engine_domain  SubClassName=ps_output  LeftPortType=input  RightPortType=output  PseudoPeriodic=off  Frequencies=[]  VectorFormat=1-D array  Unit=A  AffineConversion=off
  Vn : nesl_utility/Simulink-PS Converter  PhysicalDomain=network_engine_domain  SubClassName=ps_input  LeftPortType=input  RightPortType=output  PseudoPeriodic=off  Frequencies=[]  NoiseDistribution=none  NoiseParameters=[]  Unit=V  AffineConversion=off  FilteringAndDerivatives=zero  SimscapeFilterOrder=1  InputFilterTimeConstant=0.001  UdotUserProvided=1
  2 : PMIOPort  Side=Right
  current : Outport
  wires:
  In/1 -> current/1
  voltage/1 -> Vn/1
  connections:
  Current Sensor/RConn1 -- In/LConn1
  Electrical Reference/LConn1 -- Controlled Voltage Source/RConn2
  Current Sensor/RConn2 -- Controlled Voltage Source/LConn1
  Vn/RConn1 -- Controlled Voltage Source/RConn1
  2/RConn1 -- Current Sensor/LConn1

== system ElectricalCoupling_testing/Network Coupler (Current-Voltage)2/Port 1 Interface ==
  current : Inport
  Controlled Current Source : fl_lib/Electrical/Electrical Sources/Controlled Current Source
  Electrical Reference : fl_lib/Electrical/Electrical Elements/Electrical Reference
  Electrical Reference1 : fl_lib/Electrical/Electrical Elements/Electrical Reference
  Interface : Subsystem  Variant=on  VariantControlMode=label  VariantControl=Variant1  LabelModeActiveChoice=Continuous
      settings: PortSchema="{\"entries\":[{\"content\":{\"sides\":[{\"content\":{\"connectorIds\":[\"In1\",\"Out2\"]},\"type\":\"ConnectorPlacement.EquallySpacedRectSide\",\"uuid\":\"aa56821c-7799-44e3-b228-553c5b43a68d\"},{\"content\":{\"connectorIds\":[\"In2\",\"Out1\"],\"side\":\"RIGHT\"},\"type\":\"ConnectorPlacement.EquallySpacedRectSide\",\"uuid\":\"8658dee5-55e2-4f33-bdec-e6600ce27fc1\"},{\"content\":{\"connectorIds\":[],\"side\":\"TOP\"},\"type\":\"ConnectorPlacement.EquallySpacedRectSide\",\"uuid\":\"2effe9c6-8e61-4f0c-a39b-329d9ffc707d\"}]},\"type\":\"ConnectorPlacement.EquallySpacedConnector\",\"uuid\":\"c8fc8444-dfc7-49a5-9550-b957635f7d8f\"}],\"packageUris\":[\"http://schema.mathworks.com/mf0/Connector/R2020b\"],\"version\":\"1.0\"}"
  Ip : nesl_utility/Simulink-PS Converter  PhysicalDomain=network_engine_domain  SubClassName=ps_input  LeftPortType=input  RightPortType=output  PseudoPeriodic=off  Frequencies=[]  NoiseDistribution=none  NoiseParameters=[]  Unit=A  AffineConversion=off  FilteringAndDerivatives=zero  SimscapeFilterOrder=1  InputFilterTimeConstant=0.001  UdotUserProvided=1
  Voltage Sensor : fl_lib/Electrical/Electrical Sensors/Voltage Sensor
  Vp : nesl_utility/PS-Simulink Converter  PhysicalDomain=network_engine_domain  SubClassName=ps_output  LeftPortType=input  RightPortType=output  PseudoPeriodic=off  Frequencies=[]  VectorFormat=1-D array  Unit=V  AffineConversion=off
  1 : PMIOPort  Side=Left
  voltage : Outport
  wires:
  Interface/2(through1) -> Ip/1
  Vp/1 -> Interface/1(across1)
  current/1 -> Interface/2(through2)
  Interface/1(across2) -> voltage/1
  connections:
  Electrical Reference1/LConn1 -- Voltage Sensor/RConn2
  Ip/RConn1 -- Controlled Current Source/RConn1
  Voltage Sensor/RConn1 -- Vp/LConn1
  Controlled Current Source/LConn1 -- Electrical Reference/LConn1
  Voltage Sensor/LConn1 -- 1/RConn1 -- Controlled Current Source/RConn2

== system ElectricalCoupling_testing/Network Coupler (Current-Voltage)2/Port 2 Interface ==
  voltage : Inport
  Controlled Voltage Source : fl_lib/Electrical/Electrical Sources/Controlled Voltage Source
  Current Sensor : fl_lib/Electrical/Electrical Sensors/Current Sensor
  Electrical Reference : fl_lib/Electrical/Electrical Elements/Electrical Reference
  In : nesl_utility/PS-Simulink Converter  PhysicalDomain=network_engine_domain  SubClassName=ps_output  LeftPortType=input  RightPortType=output  PseudoPeriodic=off  Frequencies=[]  VectorFormat=1-D array  Unit=A  AffineConversion=off
  Vn : nesl_utility/Simulink-PS Converter  PhysicalDomain=network_engine_domain  SubClassName=ps_input  LeftPortType=input  RightPortType=output  PseudoPeriodic=off  Frequencies=[]  NoiseDistribution=none  NoiseParameters=[]  Unit=V  AffineConversion=off  FilteringAndDerivatives=zero  SimscapeFilterOrder=1  InputFilterTimeConstant=0.001  UdotUserProvided=1
  2 : PMIOPort  Side=Right
  current : Outport
  wires:
  voltage/1 -> Vn/1
  In/1 -> current/1
  connections:
  2/RConn1 -- Current Sensor/LConn1
  Vn/RConn1 -- Controlled Voltage Source/RConn1
  Current Sensor/RConn2 -- Controlled Voltage Source/LConn1
  Electrical Reference/LConn1 -- Controlled Voltage Source/RConn2
  Current Sensor/RConn1 -- In/LConn1

== system ElectricalCoupling_testing/Network Coupler (Current-Voltage)/Port 1 Interface/Interface ==
  across1 : Inport
  through2 : Inport  Port=2
  Continuous : Subsystem  VariantControl=Continuous
  Discrete : Subsystem  VariantControl=Discrete
  across2 : Outport
  through1 : Outport  Port=2

== system ElectricalCoupling_testing/Network Coupler (Current-Voltage)1/Port 1 Interface/Interface ==
  across1 : Inport
  through2 : Inport  Port=2
  Continuous : Subsystem  VariantControl=Continuous
  Discrete : Subsystem  VariantControl=Discrete
  across2 : Outport
  through1 : Outport  Port=2

== system ElectricalCoupling_testing/Network Coupler (Current-Voltage)2/Port 1 Interface/Interface ==
  across1 : Inport
  through2 : Inport  Port=2
  Continuous : Subsystem  VariantControl=Continuous
  Discrete : Subsystem  VariantControl=Discrete
  across2 : Outport
  through1 : Outport  Port=2

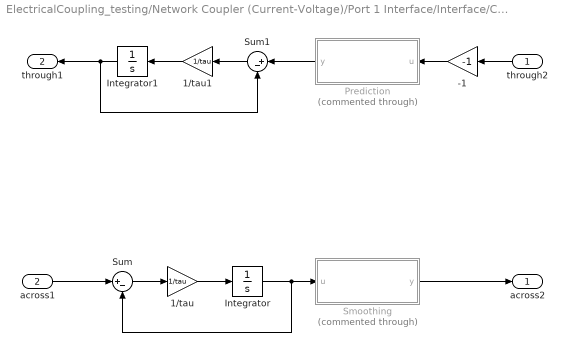
== system ElectricalCoupling_testing/Network Coupler (Current-Voltage)/Port 1 Interface/Interface/Continuous ==
  through2 : Inport
  across1 : Inport  Port=2
  -1 : Gain  Gain=-1  SaturateOnIntegerOverflow=on  OutDataTypeStr=Inherit: Same as input  ParamDataTypeStr=Inherit: Same as input
  1/tau : Gain  Gain=1/tau  SaturateOnIntegerOverflow=on  OutDataTypeStr=Inherit: Same as input  ParamDataTypeStr=Inherit: Same as input
  1/tau1 : Gain  Gain=1/tau  SaturateOnIntegerOverflow=on  OutDataTypeStr=Inherit: Same as input  ParamDataTypeStr=Inherit: Same as input
  Integrator : Integrator  InitialCondition=v0
  Integrator1 : Integrator  InitialCondition=i0
  Prediction : Subsystem  Commented=through  mask(Prediction (discrete->continuous)){h2=h2}
      mask prompts: h2 "physmod:simscape:couplers:SimscapeNetworkCouplersLib:PortUDiscreteSampleTimes_MP"
      mask help: physmod:simscape:couplers:SimscapeNetworkCouplersLib:Predictiondiscretecontinuous_MD
      mask DialogControl h2 Prompt: Port u discrete sample time (s)
  Smoothing : Subsystem  Commented=through  mask(Smoothing (continuous->discrete)){tsSmoothing=tsSmoothing, smoothing0=v0}
      mask prompts: tsSmoothing "physmod:simscape:couplers:SimscapeNetworkCouplersLib:SmoothingTimeConstants_MP"; smoothing0 "physmod:simscape:couplers:SimscapeNetworkCouplersLib:InitialOutput_MP"
      mask help: physmod:simscape:couplers:SimscapeNetworkCouplersLib:Smoothingcontinuousdiscrete_MD
      mask DialogControl tsSmoothing Prompt: Smoothing time constant (s)
      mask DialogControl smoothing0 Prompt: Initial output
  Sum : Sum  Inputs=|+-  InputSameDT=on  SaturateOnIntegerOverflow=on  OutDataTypeStr=Inherit: Same as first input
  Sum1 : Sum  Inputs=|+-  InputSameDT=on  SaturateOnIntegerOverflow=on  OutDataTypeStr=Inherit: Same as first input
  across2 : Outport
  through1 : Outport  Port=2
  wires:
  Smoothing/1(y) -> across2/1
  -1/1 -> Prediction/1(u)
  through2/1 -> -1/1
  1/tau/1 -> Integrator/1
  Sum/1 -> 1/tau/1
  Integrator/1 -> Sum/2, Smoothing/1(u)
  across1/1 -> Sum/1
  Integrator1/1 -> Sum1/2, through1/1
  1/tau1/1 -> Integrator1/1
  Sum1/1 -> 1/tau1/1
  Prediction/1(y) -> Sum1/1
